simulink model "vsg_stage5k_tx9_ff08"  (R2018b)
settings: Solver=ode23tb  StartTime=0.0  StopTime=11  MaxStep=2.5e-06  RelTol=1e-4  AbsTol=1e-6
model workspace (MAT data in the model file):
  e12_lpf_K = 0.385869545095
  secondary_Ts = 0.0001
  secondary_enable_time = 0.5
  secondary_max_pu = 0.8
  secondary_min_pu = -0.5
  vsg_D = 0.5
  vsg_Dq = 0.007
  vsg_H = 5
  vsg_L_load = 0.001
  vsg_P_set_pu = 1
  vsg_Q_set = 0
  vsg_R_load = 1587
  vsg_R_step = 680.142857143
  vsg_Rp = 0.05
  vsg_S = 100
  vsg_Vdc_floor = 10
  vsg_Vdc_t = [0 1]
  vsg_Vdc_v = [48 48]
  vsg_Vrms = 10.4706499426
  vsg_duty_max = 0.97
  vsg_duty_min = 0.03
  vsg_f0 = 50
  vsg_f_lpf_PQ = 5
  vsg_ff_on = 0.8
  vsg_fsw = 20000
  vsg_secondary_Ki = 4
  vsg_secondary_on = 1
  vsg_t_softstart = 0.1
  vsg_t_step_down = 7
  vsg_t_step_up = 3
  vsg_tx_Pn = [50 50]
  vsg_tx_RmLm = [33.3333333333 9.09090909091]
  vsg_tx_w1 = [9.9 0.041154606648 0.0123463819944]
  vsg_tx_w2 = [230 0.041154606648 0.0123463819944]
undefined symbols (not defined in the file): DiscIntNeverNeededParam
libraries: powerlib x49, simulink x5
(part 2 of 2)

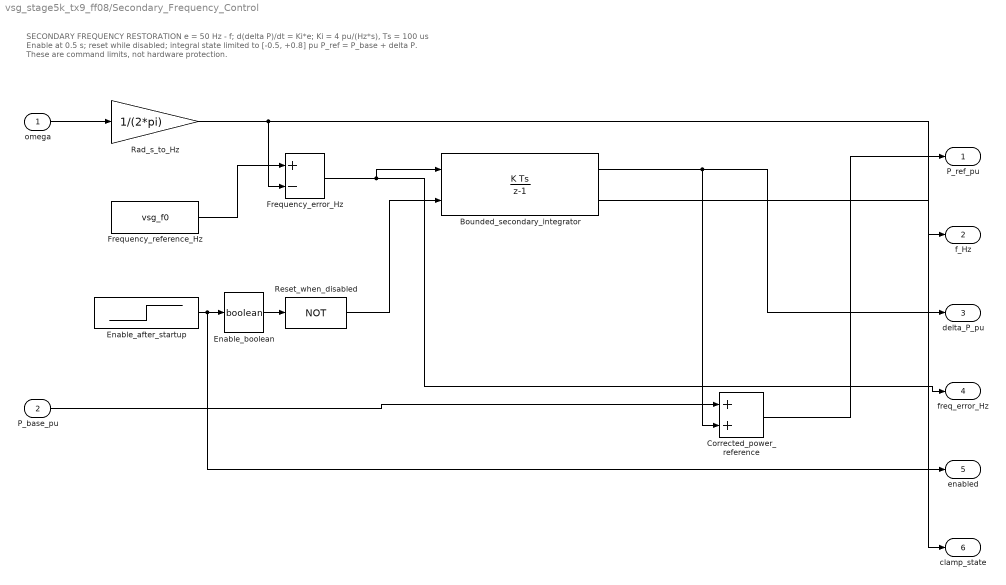
== system vsg_stage5k_tx9_ff08/Secondary_Frequency_Control ==
  note: SECONDARY FREQUENCY RESTORATION
      | e = 50 Hz - f; d(delta P)/dt = Ki*e; Ki = 4 pu/(Hz*s), Ts = 100 us
      | Enable at 0.5 s; reset while disabled; integral state limited to [-0.5, +0.8] pu
      | P_ref = P_base + delta P. These are command limits, not hardware protection.
  omega : Inport
  P_base_pu : Inport  Port=2
  Bounded_secondary_integrator : DiscreteIntegrator  gainval=vsg_secondary_Ki  ExternalReset=level  SampleTime=secondary_Ts  LimitOutput=on  UpperSaturationLimit=secondary_max_pu  LowerSaturationLimit=secondary_min_pu  ShowSaturationPort=on  ICPrevOutput=DiscIntNeverNeededParam  ICPrevScaledInput=DiscIntNeverNeededParam
  Corrected_power_reference : Sum  SaturateOnIntegerOverflow=on  InputSameDT=on  OutDataTypeStr=Inherit: Same as first input
  Enable_after_startup : Step  Time=secondary_enable_time  After=vsg_secondary_on  SampleTime=secondary_Ts
  Enable_boolean : DataTypeConversion  OutDataTypeStr=boolean  SaturateOnIntegerOverflow=on  RndMeth=Zero
  Frequency_error_Hz : Sum  Inputs=+-  SaturateOnIntegerOverflow=on  InputSameDT=on  OutDataTypeStr=Inherit: Same as first input
  Frequency_reference_Hz : Constant  Value=vsg_f0
  Rad_s_to_Hz : Gain  Gain=1/(2*pi)  SaturateOnIntegerOverflow=on  OutDataTypeStr=Inherit: Same as input  ParamDataTypeStr=Inherit: Same as input
  Reset_when_disabled : Logic  Operator=NOT
  P_ref_pu : Outport
  f_Hz : Outport  Port=2
  delta_P_pu : Outport  Port=3
  freq_error_Hz : Outport  Port=4
  enabled : Outport  Port=5
  clamp_state : Outport  Port=6
  wires:
  omega/1 -> Rad_s_to_Hz/1
  Frequency_reference_Hz/1 -> Frequency_error_Hz/1
  Rad_s_to_Hz/1 -> Frequency_error_Hz/2, f_Hz/1
  Enable_after_startup/1 -> Enable_boolean/1, enabled/1
  Enable_boolean/1 -> Reset_when_disabled/1
  Frequency_error_Hz/1 -> Bounded_secondary_integrator/1, freq_error_Hz/1
  Reset_when_disabled/1 -> Bounded_secondary_integrator/2
  P_base_pu/1 -> Corrected_power_reference/1
  Bounded_secondary_integrator/1 -> Corrected_power_reference/2, delta_P_pu/1
  Corrected_power_reference/1 -> P_ref_pu/1
  Bounded_secondary_integrator/2 -> clamp_state/1
